simulink model "nl_gain_antenna"  (R2025b)
settings: Solver=ode45  StartTime=0.0  StopTime=10  MaxStep=1e-3  RelTol=1e-3
values from neighbouring files (symbols this model uses):
  am = 1.71    [nl_gain_demo.m]
  c2 = 0.2083    [nl_gain_demo.m]
  Kd = 15    [nl_gain_demo.m]    (also in pVsScheduledPd.m)
  Kfar = 300    [nl_gain_demo.m]    (also in pVsScheduledPd.m)
  Knear = 60    [nl_gain_demo.m]    (also in pVsScheduledPd.m)
  kpot = 0.318    [nl_gain_demo.m]
  V0 = 0.318    [nl_gain_demo.m]
  Vi = 1    [fan_out.m]    (also in nl_gain_demo.m; one_volt.m; pVsScheduledPd.m)
settings Model: Creator=Lenovo  LastModifiedBy=Lenovo

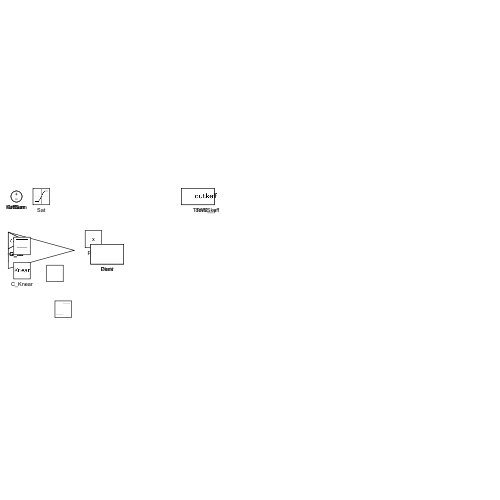
[thumbnail: Simulink's stored preview of the top-level diagram]
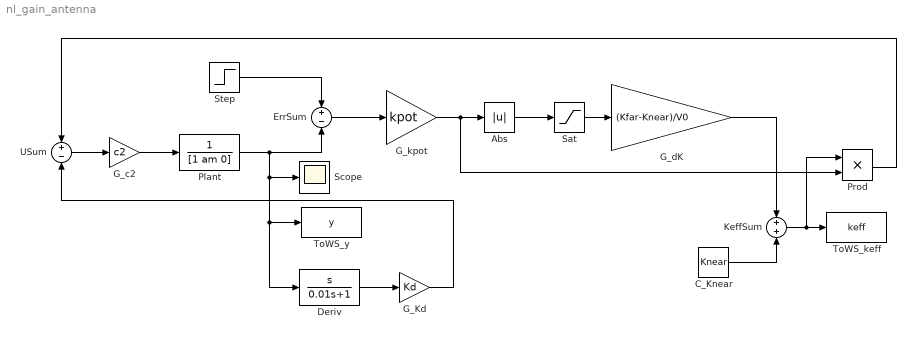
== system nl_gain_antenna ==
  Abs : Abs  SaturateOnIntegerOverflow=off
  C_Knear : Constant  Value=Knear
  Deriv : TransferFcn  Numerator=[1 0]  Denominator=[0.01 1]
  ErrSum : Sum  Inputs=+-
  G_Kd : Gain  Gain=Kd
  G_c2 : Gain  Gain=c2
  G_dK : Gain  Gain=(Kfar-Knear)/V0
  G_kpot : Gain  Gain=kpot
  KeffSum : Sum
  Plant : TransferFcn  Numerator=1  Denominator=[1 am 0]
  Prod : Product
  Sat : Saturate  UpperLimit=V0  LowerLimit=0
  Scope : Scope
  Step : Step  Time=0  After=Vi  SampleTime=0
  ToWS_keff : ToWorkspace  VariableName=keff  SaveFormat=Timeseries  SampleTime=-1
  ToWS_y : ToWorkspace  VariableName=y  SaveFormat=Timeseries  SampleTime=-1
  USum : Sum  Inputs=+-
  wires:
  G_Kd/1 -> USum/2
  Plant/1 -> Deriv/1, ToWS_y/1, Scope/1, ErrSum/2
  USum/1 -> G_c2/1
  Deriv/1 -> G_Kd/1
  G_c2/1 -> Plant/1
  Step/1 -> ErrSum/1
  G_kpot/1 -> Prod/2, Abs/1
  ErrSum/1 -> G_kpot/1
  Abs/1 -> Sat/1
  Sat/1 -> G_dK/1
  Prod/1 -> USum/1
  G_dK/1 -> KeffSum/1
  C_Knear/1 -> KeffSum/2
  KeffSum/1 -> Prod/1, ToWS_keff/1
